simulink library "ConverterLibrary"  (R2026a)
settings: Solver=VariableStepAuto
undefined symbols (not defined in the file or in its folder): DiscIntNeverNeededParam, dspblkCoreblockFVToolHelper, gcbh, gridInverter
libraries: fl_lib x240, nesl_utility x221, ee_lib x208, slpidlib x28, eeGeneralControl x12, simulink x9, eeTransforms x4, simulink_extras x1, eePowerMeasurement x1
(part 4 of 30)

== system ConverterLibrary/Power Converter Plant/Soft-Switching Converters ==
  CLLC Converter : Subsystem  mask(CLLC Converter Plant){modelOption=Simplified, C1=6.9269e-7, C1_unit=F, Rcr1=0.001, Rcr1_unit=Ohm, C2=7.487e-7, C2_unit=F, Rcr2=0.001, Rcr2_unit=Ohm, Llk1=3.6568e-6, Llk1_unit=H, R1=0.01, R1_unit=Ohm, Llk2=3.3829e-6, Llk2_unit=H, R2=0.01, R2_unit=Ohm, Lm=5.4852e-5, Lm_unit=H, N1=30, N2=29, Co=1.0667e-3, Co_unit=F, Rco=0.02, Rco_unit=Ohm, Vco=350, Vco_unit=V, PrimaryDeviceOption=MOSFET (Ideal, Switching) with Thermal, PrimaryRon=0.001, PrimaryRon_unit=Ohm, PrimaryGoff=1e-5, PrimaryGoff_unit=1/Ohm, PrimaryVth=2.5, PrimaryVth_unit=V, PrimaryVbodydiodeOn=0.6, PrimaryVbodydiodeOn_unit=V, PrimaryRbodydiodeOn=0.001, PrimaryRbodydiodeOn_unit=Ohm, PrimaryGbodydiodeOff=1e-5, PrimaryGbodydiodeOff_unit=1/Ohm, PrimaryCparasitic=2e-10, PrimaryCparasitic_unit=F, SecondaryDeviceOption=MOSFET (Ideal, Switching) with Thermal, SecondaryRon=0.001, SecondaryRon_unit=Ohm, SecondaryGoff=1e-5, SecondaryGoff_unit=1/Ohm, SecondaryVth=2.5, SecondaryVth_unit=V, SecondaryVbodydiodeOn=0.6, SecondaryVbodydiodeOn_unit=V, SecondaryRbodydiodeOn=0.001, SecondaryRbodydiodeOn_unit=Ohm, SecondaryGbodydiodeOff=1e-5, SecondaryGbodydiodeOff_unit=1/Ohm, SecondaryCparasitic=2e-10, SecondaryCparasitic_unit=F, PrimarySimTemp=25, PrimarySimTemp_unit=degC, SecondarySimTemp=25, SecondarySimTemp_unit=degC}
      mask prompts: modelOption "Model option"; C1 "Primary resonant capacitance (C1)"; Rcr1 "Primary resonant capacitor ESR (Rcr1)"; C2 "Secondary resonant capacitance (C2)"; Rcr2 "Secondary resonant capacitor ESR (Rcr2)"; Llk1 "Primary leakage inductance (Llk1)"; R1 "Primary resistance (R1)"; Llk2 "Secondary leakage inductance (Llk2)"; R2 "Secondary resistance (R2)"; Lm "Magnetizing inductance (Lm)"; N1 "Transformer primary number of turns (N1)"; N2 "Transformer secondary number of turns (N2)"; Co "Secondary output capacitance (Co)"; Rco "Secondary output capacitance ESR (Rco)"; Vco "Initial output capacitor voltage"; PrimaryDeviceOption "Select the primary switching device"; PrimaryRon "On-state resistance"; PrimaryGoff "Off-state conductance"; PrimaryVth "Threshold voltage"; PrimaryVbodydiodeOn "Body diode forward voltage"; PrimaryRbodydiodeOn "Body diode on-resistance"; PrimaryGbodydiodeOff "Body diode off-conductance"; PrimaryCparasitic "MOSFET parasitic capacitance"; SecondaryDeviceOption "Select the secondary switching device"; SecondaryRon "On-state resistance"; SecondaryGoff "Off-state conductance"; SecondaryVth "Threshold voltage"; SecondaryVbodydiodeOn "Body diode forward voltage"; SecondaryRbodydiodeOn "Body diode on-resistance"; SecondaryGbodydiodeOff "Body diode off-conductance"; SecondaryCparasitic "MOSFET parasitic capacitance"; PrimarySimTemp "Simulation temperature"; SecondarySimTemp "Simulation temperature"
      mask help: This block models the power circuit of the CLLC resonant converter. You can choose between different semicondcutor switch model for primary and secondaryconverter. You can choose between ideal semiconductor switch, MOSFET without thermal port and tabulated MOSFET with thermal port.
      mask init:
      | %% Unit conversion: convert displayed values to base SI units
      | convMap = containers.Map( ...
      |     {'W','kW','MW','V','kV','mV','F','mF','uF','nF','pF', ...
      |      'H','mH','uH','nH','Ohm','kOhm','mOhm','S','mS','1/Ohm'}, ...
      |     {1, 1e3, 1e6, 1, 1e3, 1e-3, 1, 1e-3, 1e-6, 1e-9, 1e-12, ...
      |      1, 1e-3, 1e-6, 1e-9, 1, 1e3, 1e-3, 1, 1e-3, 1});
      | C1 = C1 * convMap(C1_unit);
      | Rcr1 = Rcr1 * convMap(Rcr1_unit);
      | C2 = C2 * convMap(C2_unit);
      | Rcr2 = Rcr2 * convMap(Rcr2_unit);
      | Llk1 = Llk1 * convMap(Llk1_unit);
      | R1 = R1 * convMap(R1_unit);
      | Llk2 = Llk2 * convMap(Llk2_unit);
      | R2 = R2 * convMap(R2_unit);
      | Lm = Lm * convMap(Lm_unit);
      | Co = Co * convMap(Co_unit);
      | Rco = Rco * convMap(Rco_unit);
      | Vco = Vco * convMap(Vco_unit);
      | PrimaryRon = PrimaryRon * convMap(PrimaryRon_unit);
      | PrimaryGoff = PrimaryGoff * convMap(PrimaryGoff_unit);
      | PrimaryVth = PrimaryVth * convMap(PrimaryVth_unit);
      | PrimaryVbodydiodeOn = PrimaryVbodydiodeOn * convMap(PrimaryVbodydiodeOn_unit);
      | PrimaryRbodydiodeOn = PrimaryRbodydiodeOn * convMap(PrimaryRbodydiodeOn_unit);
      | PrimaryGbodydiodeOff = PrimaryGbodydiodeOff * convMap(PrimaryGbodydiodeOff_unit);
      | PrimaryCparasitic = PrimaryCparasitic * convMap(PrimaryCparasitic_unit);
      | SecondaryRon = SecondaryRon * convMap(SecondaryRon_unit);
      | SecondaryGoff = SecondaryGoff * convMap(SecondaryGoff_unit);
      | SecondaryVth = SecondaryVth * convMap(SecondaryVth_unit);
      | SecondaryVbodydiodeOn = SecondaryVbodydiodeOn * convMap(SecondaryVbodydiodeOn_unit);
      | SecondaryRbodydiodeOn = SecondaryRbodydiodeOn * convMap(SecondaryRbodydiodeOn_unit);
      | SecondaryGbodydiodeOff = SecondaryGbodydiodeOff * convMap(SecondaryGbodydiodeOff_unit);
      | SecondaryCparasitic = SecondaryCparasitic * convMap(SecondaryCparasitic_unit);
      | % Simulation temperature (primary bridge, thermal MOSFETs)
      | % Temperature is an OFFSET unit (K = degC + 273.15), so it cannot use the
      | % multiplicative convMap above; convert it explicitly. PrimarySimTemp_K is read directly
      | % by each primary thermal MOSFET junction-temperature initial target and by every
      | % Temperature Source in the primary bridge.
      | if strcmp(PrimarySimTemp_unit, 'degC')
      |     PrimarySimTemp_K = PrimarySimTemp + 273.15;
      | elseif strcmp(PrimarySimTemp_unit, 'K')
      |     PrimarySimTemp_K = PrimarySimTemp;
      | else
      |     error('CLLC Converter Power Circuit: unrecognized simulation-temperature unit "%s" (expected degC or K).', PrimarySimTemp_unit);
      | end
      | % Simulation temperature (secondary bridge, thermal MOSFETs)
      | % Temperature is an OFFSET unit (K = degC + 273.15), so it cannot use the
      | % multiplicative convMap above; convert it explicitly. SecondarySimTemp_K is read directly
      | % by each secondary thermal MOSFET junction-temperature initial target and by every
      | % Temperature Source in the secondary bridge.
      | if strcmp(SecondarySimTemp_unit, 'degC')
      |     SecondarySimTemp_K = SecondarySimTemp + 273.15;
      | elseif strcmp(SecondarySimTemp_unit, 'K')
      |     SecondarySimTemp_K = SecondarySimTemp;
      | else
      |     error('CLLC Converter Power Circuit: unrecognized simulation-temperature unit "%s" (expected degC or K).', SecondarySimTemp_unit);
      | end
      settings: CopyFcn="set_param(gcbh,\"LinkStatus\",\"none\");"  PortSchema="{\"entries\":[{\"content\":{\"sides\":[{\"content\":{\"connectorIds\":[\"LConn1\",\"LConn2\"]},\"type\":\"ConnectorPlacement.EquallySpacedRectSide\",\"uuid\":\"0e984043-8111-4613-9feb-f4d4d19f792a\"},{\"content\":{\"connectorIds\":[\"RConn1\",\"RConn2\"],\"side\":\"RIGHT\"},\"type\":\"ConnectorPlacement.EquallySpacedRectSide\",\"uuid\":\"aee9207a-aaf7-4114-a348-153041cb19a5\"},{\"content\":{\"connectorIds\":[\"In1\",\"Out1\",\"In2\"],\"side\":\"TOP\"},\"type\":\"ConnectorPlacement.EquallySpacedRectSide\",\"uuid\":\"cf17a722-cb18-4642-bf19-4f4ee8ce3a25\"}]},\"type\":\"ConnectorPlacement.EquallySpacedConnector\",\"uuid\":\"0a50e5d5-a4bf-4817-9816-42fb9bad860d\"}],\"packageUris\":[\"http://schema.mathworks.com/mf0/Connector/R2020b\"],\"version\":\"1.0\"}"
      mask Help: web('CLLCPowerCircuit.html')
      mask TypeOptions modelOption: Simplified | Detailed
      mask Callback modelOption: selectCLLCConverterModelOption(gcb);
      mask TypeOptions C1_unit: F | mF | uF | nF | pF
      mask TypeOptions Rcr1_unit: Ohm | kOhm | mOhm
      mask TypeOptions C2_unit: F | mF | uF | nF | pF
      mask TypeOptions Rcr2_unit: Ohm | kOhm | mOhm
      mask TypeOptions Llk1_unit: H | mH | uH | nH
      mask TypeOptions R1_unit: Ohm | kOhm | mOhm
      mask TypeOptions Llk2_unit: H | mH | uH | nH
      mask TypeOptions R2_unit: Ohm | kOhm | mOhm
      mask TypeOptions Lm_unit: H | mH | uH | nH
      mask TypeOptions Co_unit: F | mF | uF | nF | pF
      mask TypeOptions Rco_unit: Ohm | kOhm | mOhm
      mask TypeOptions Vco_unit: V | kV | mV
      mask TypeOptions PrimaryDeviceOption: Ideal Switch | MOSFET (Ideal, Switching) with Thermal
      mask Callback PrimaryDeviceOption: selectCLLCPrimaryMOSFET(gcb);
      mask TypeOptions PrimaryRon_unit: Ohm | kOhm | mOhm
      mask TypeOptions PrimaryGoff_unit: 1/Ohm | S | mS
      mask TypeOptions PrimaryVth_unit: V | kV | mV
      mask TypeOptions PrimaryVbodydiodeOn_unit: V | mV
      mask TypeOptions PrimaryRbodydiodeOn_unit: Ohm | kOhm | mOhm
      mask TypeOptions PrimaryGbodydiodeOff_unit: 1/Ohm | S | mS
      mask TypeOptions PrimaryCparasitic_unit: F | mF | uF | nF | pF
      mask TypeOptions SecondaryDeviceOption: Ideal Switch | MOSFET (Ideal, Switching) with Thermal
      mask Callback SecondaryDeviceOption: selectCLLCSecondaryMOSFET(gcb);
      mask TypeOptions SecondaryRon_unit: Ohm | kOhm | mOhm
      mask TypeOptions SecondaryGoff_unit: 1/Ohm | S | mS
      mask TypeOptions SecondaryVth_unit: V | kV | mV
      mask TypeOptions SecondaryVbodydiodeOn_unit: V | mV
      mask TypeOptions SecondaryRbodydiodeOn_unit: Ohm | kOhm | mOhm
      mask TypeOptions SecondaryGbodydiodeOff_unit: 1/Ohm | S | mS
      mask TypeOptions SecondaryCparasitic_unit: F | mF | uF | nF | pF
      mask TypeOptions PrimarySimTemp_unit: degC | K
      mask TypeOptions SecondarySimTemp_unit: degC | K
      mask DialogControl ParameterGroupVar Prompt: CLLC Resonant Converter Plant
      mask DialogControl CLLCTank Prompt: CLLC converter parameters
      mask DialogControl TransformerParameters Prompt: Transformer
      mask DialogControl PrimarySwitch Prompt: Primary semiconductor switch
      mask DialogControl PrimaryOpenMOSFETMask Prompt: Open the MOSFET block mask
      mask DialogControl PrimaryOpenMOSFETMask Callback: openCLLCDeviceMask(gcb, 'primaryThermalMOSFET');
      mask DialogControl PrimaryApplyMOSFETParam Prompt: Apply parameters to all primary MOSFET blocks
      mask DialogControl PrimaryApplyMOSFETParam Callback: applyCLLCDeviceParameters(gcb, 'primaryThermalMOSFET');
      mask DialogControl SecondarySwitch Prompt: Secondary semiconductor switch
      mask DialogControl SecondaryOpenMOSFETMask Prompt: Open the MOSFET block mask
      mask DialogControl SecondaryOpenMOSFETMask Callback: openCLLCDeviceMask(gcb, 'secondaryThermalMOSFET');
      mask DialogControl SecondaryApplyMOSFETParam Prompt: Apply parameters to all secondary MOSFET blocks
      mask DialogControl SecondaryApplyMOSFETParam Callback: applyCLLCDeviceParameters(gcb, 'secondaryThermalMOSFET');
      mask DialogControl ExportPanel Prompt: Export to Unmasked Subsystem
      mask DialogControl ExportInfo Prompt: To customize the converter, export it as an unmasked subsystem with the active variant flattened - a standalone, fully-editable circuit plus a parameter file. Requires the "Variant Manager for Simulink" add-on.
      mask DialogControl exportToModel Prompt: Export
      mask DialogControl exportToModel Callback: exportConverterModelFromMask(gcb);
      mask Display: image('CLLCConverterIcon.svg');
  DAB Converter : Subsystem  mask(Dual Active Bridge DC-DC Converter){modelOption=Detailed, ratedPower=10000, ratedPower_unit=W, Vin=750, Vin_unit=V, Vout=525, Vout_unit=V, Fsw=100000, Fsw_unit=Hz, turnsRatio=1.4286, Co=2.963e-5, Co_unit=F, Rco=1, Rco_unit=mOhm, seriesInductorOption=Use transformer leakage inductance, Lr=0, Lr_unit=H, RLr=0.01, RLr_unit=Ohm, Lm=1.4062e-3, Lm_unit=H, Llk1=3.913e-5, Llk1_unit=H, RLlk1=0.01, RLlk1_unit=Ohm, Llk2=4.7935e-6, Llk2_unit=H, RLlk2=0.01, RLlk2_unit=Ohm, Vco=525, Vco_unit=V, switchDeviceOptionPri=MOSFET (Ideal, Switching) with Thermal, RdsOnPri=0.005, RdsOnPri_unit=Ohm, GdsOffPri=1e-5, GdsOffPri_unit=1/Ohm, VthPri=3, VthPri_unit=V, CossPri=2e-10, CossPri_unit=F, simTempPri=25, simTempPri_unit=degC, VfPri=0.005, VfPri_unit=V, RdPri=1, RdPri_unit=mOhm, GdPri=1e-5, GdPri_unit=1/Ohm, switchDeviceOptionSec=MOSFET (Ideal, Switching) with Thermal, RdsOnSec=0.005, RdsOnSec_unit=Ohm, GdsOffSec=1e-5, GdsOffSec_unit=1/Ohm, VthSec=3, VthSec_unit=V, CossSec=2e-10, CossSec_unit=F, simTempSec=25, simTempSec_unit=degC, VfSec=0.005, VfSec_unit=V, RdSec=1, RdSec_unit=mOhm, GdSec=1e-5, GdSec_unit=1/Ohm}
      mask prompts: modelOption "Model option"; ratedPower "Rated power"; Vin "Nominal input voltage"; Vout "Nominal output voltage"; Fsw "Switching frequency"; turnsRatio "Transformer turns ratio (Np/Ns)"; Co "Secondary output capacitance"; Rco "Secondary output capacitance ESR"; seriesInductorOption "Series inductance"; Lr "Series inductance (Lr)"; RLr "Series inductance resistance"; Lm "Magnetizing inductance (Lm)"; Llk1 "Primary leakage inductance (Llk1)"; RLlk1 "Primary winding resistance"; Llk2 "Secondary leakage inductance (Llk2)"; RLlk2 "Secondary winding resistance"; Vco "Initial output capacitor voltage"; switchDeviceOptionPri "Switch device"; RdsOnPri "On-state resistance (RdsOn)"; GdsOffPri "Off-state conductance (GdsOff)"; VthPri "Threshold voltage"; CossPri "Output capacitance (Coss)"; simTempPri "Simulation temperature"; VfPri "Diode forward voltage (Vf)"; RdPri "Diode on resistance (Rd)"; GdPri "Diode off conductance (Gd)"; switchDeviceOptionSec "Switch device"; RdsOnSec "On-state resistance (RdsOn)"; GdsOffSec "Off-state conductance (GdsOff)"; VthSec "Threshold voltage"; CossSec "Output capacitance (Coss)"; simTempSec "Simulation temperature"; VfSec "Diode forward voltage (Vf)"; RdSec "Diode on resistance (Rd)"; GdSec "Diode off conductance (Gd)"
      mask help: Dual Active Bridge (DAB) DC-DC Converter with variant options for HDL and Simulation models.
      mask init:
      | %% Unit conversion: convert displayed values to base SI units
      | convMap = containers.Map( ...
      |     {'W','kW','MW','V','kV','mV','F','mF','uF','nF','pF', ...
      |      'H','mH','uH','nH','Ohm','kOhm','mOhm','S','mS','1/Ohm', ...
      |      'Hz','kHz','MHz'}, ...
      |     {1, 1e3, 1e6, 1, 1e3, 1e-3, 1, 1e-3, 1e-6, 1e-9, 1e-12, ...
      |      1, 1e-3, 1e-6, 1e-9, 1, 1e3, 1e-3, 1, 1e-3, 1, ...
      |      1, 1e3, 1e6});
      | 
      | ratedPower_SI = ratedPower * convMap(ratedPower_unit);
      | Vin_SI = Vin * convMap(Vin_unit);
      | Vout_SI = Vout * convMap(Vout_unit);
      | Fsw_SI = Fsw * convMap(Fsw_unit);
      | Llk1_SI = Llk1 * convMap(Llk1_unit);
      | RLlk1_SI = RLlk1 * convMap(RLlk1_unit);
      | Llk2_SI = Llk2 * convMap(Llk2_unit);
      | RLlk2_SI = RLlk2 * convMap(RLlk2_unit);
      | Lr_SI = Lr * convMap(Lr_unit);
      | RLr_SI = RLr * convMap(RLr_unit);
      | % When the model compiles, the transformer leakages must be positive, and so must Lr when the
      | % external inductor is used. A dialog change is not checked, so Lr can be entered after the option.
      | if any(strcmp(get_param(bdroot(gcb), 'SimulationStatus'), {'updating', 'initializing'}))
      |     if ~(isfinite(Llk1_SI) && Llk1_SI > 0 && isfinite(Llk2_SI) && Llk2_SI > 0)
      |         error('The transformer leakage inductances must be positive. Primary: %g H, secondary: %g H.', Llk1_SI, Llk2_SI);
      |     end
      |     if strcmp(get_param(gcb, 'seriesInductorOption'), 'Use external inductance') && ~(isfinite(Lr_SI) && Lr_SI > 0)
      |         error('The external series inductance must be positive when it is used. Lr: %g H.', Lr_SI);
      |     end
      | end
      | Lm_SI = Lm * convMap(Lm_unit);
      | Co_SI = Co * convMap(Co_unit);
      | Rco_SI = Rco * convMap(Rco_unit);
      | Vco_SI = Vco * convMap(Vco_unit);
      | 
      | %% Primary switch params
      | RdsOnPri_SI = RdsOnPri * convMap(RdsOnPri_unit);
      | GdsOffPri_SI = GdsOffPri * convMap(GdsOffPri_unit);
      | VthPri_SI = VthPri * convMap(VthPri_unit);
      | CossPri_SI = CossPri * convMap(CossPri_unit);
      | 
      | %% Secondary switch params
      | RdsOnSec_SI = RdsOnSec * convMap(RdsOnSec_unit);
      | GdsOffSec_SI = GdsOffSec * convMap(GdsOffSec_unit);
      | VthSec_SI = VthSec * convMap(VthSec_unit);
      | CossSec_SI = CossSec * convMap(CossSec_unit);
      | 
      | %% Primary switch protection-diode params
      | VfPri_SI = VfPri * convMap(VfPri_unit);
      | RdPri_SI = RdPri * convMap(RdPri_unit);
      | GdPri_SI = GdPri * convMap(GdPri_unit);
      | 
      | %% Secondary switch protection-diode params
      | VfSec_SI = VfSec * convMap(VfSec_unit);
      | RdSec_SI = RdSec * convMap(RdSec_unit);
      | GdSec_SI = GdSec * convMap(GdSec_unit);
      | 
      | 
      | %% Simulation temperature (thermal MOSFET)
      | % Temperature is an OFFSET unit (K = degC + 273.15), so it cannot use the
      | % multiplicative convMap; convert it explicitly. These Kelvin variables are
      | % read directly by each thermal MOSFET device junction-temperature target and
      | % by each bridge Temperature Source.
      | if strcmp(simTempPri_unit, 'degC')
      |     simTempPri_K = simTempPri + 273.15;
      | else
      |     simTempPri_K = simTempPri;
      | end
      | if strcmp(simTempSec_unit, 'degC')
      |     simTempSec_K = simTempSec + 273.15;
      | else
      |     simTempSec_K = simTempSec;
      | end
      | 
      | %% Apply variant selection
      | selectDABConverterModelOption(gcb);
      settings: CopyFcn="set_param(gcbh,\"LinkStatus\",\"none\");"  PortSchema="{\"entries\":[{\"content\":{\"sides\":[{\"content\":{\"connectorIds\":[\"LConn1\",\"LConn2\"]},\"type\":\"ConnectorPlacement.EquallySpacedRectSide\",\"uuid\":\"5eb81d01-b33d-480d-b92b-9ee197a9667d\"},{\"content\":{\"connectorIds\":[\"RConn1\",\"RConn2\"],\"side\":\"RIGHT\"},\"type\":\"ConnectorPlacement.EquallySpacedRectSide\",\"uuid\":\"a719554b-e33a-474b-8c80-408706add5ae\"},{\"content\":{\"connectorIds\":[\"In1\",\"Out1\",\"In2\"],\"side\":\"TOP\"},\"type\":\"ConnectorPlacement.EquallySpacedRectSide\",\"uuid\":\"aea510b9-aefe-49d3-b91f-0f6ebd0a6b41\"}]},\"type\":\"ConnectorPlacement.EquallySpacedConnector\",\"uuid\":\"00bcdd44-1110-449b-876a-23d9733cbf45\"}],\"packageUris\":[\"http://schema.mathworks.com/mf0/Connector/R2020b\"],\"version\":\"1.0\"}"
      mask Help: web('DABConverter.html')
      mask TypeOptions modelOption: Simplified | Detailed
      mask Callback modelOption: selectDABConverterModelOption(gcb);
      mask TypeOptions ratedPower_unit: W | kW | MW
      mask TypeOptions Vin_unit: mV | V | kV
      mask TypeOptions Vout_unit: mV | V | kV
      mask TypeOptions Fsw_unit: Hz | kHz | MHz
      mask TypeOptions Co_unit: F | mF | uF | nF | pF
      mask TypeOptions Rco_unit: mOhm | Ohm | kOhm
      mask TypeOptions seriesInductorOption: Use external inductance | Use transformer leakage inductance
      mask Callback seriesInductorOption: selectDABSeriesInductor(gcb);
      mask TypeOptions Lr_unit: H | mH | uH | nH
      mask TypeOptions RLr_unit: mOhm | Ohm | kOhm
      mask TypeOptions Lm_unit: H | mH | uH | nH
      mask TypeOptions Llk1_unit: H | mH | uH | nH
      mask TypeOptions RLlk1_unit: mOhm | Ohm | kOhm
      mask TypeOptions Llk2_unit: H | mH | uH | nH
      mask TypeOptions RLlk2_unit: mOhm | Ohm | kOhm
      mask TypeOptions Vco_unit: V | kV | mV
      mask TypeOptions switchDeviceOptionPri: Ideal Switch | MOSFET (Ideal, Switching) with Thermal
      mask Callback switchDeviceOptionPri: selectDABConverterSwitchDevice(gcb)
      mask TypeOptions RdsOnPri_unit: mOhm | Ohm | kOhm
      mask TypeOptions GdsOffPri_unit: S | mS | 1/Ohm
      mask TypeOptions VthPri_unit: mV | V | kV
      mask TypeOptions CossPri_unit: F | mF | uF | nF | pF
      mask TypeOptions simTempPri_unit: degC | K
      mask TypeOptions VfPri_unit: mV | V | kV
      mask TypeOptions RdPri_unit: mOhm | Ohm | kOhm
      mask TypeOptions GdPri_unit: S | mS | 1/Ohm
      mask TypeOptions switchDeviceOptionSec: Ideal Switch | MOSFET (Ideal, Switching) with Thermal
      mask Callback switchDeviceOptionSec: selectDABConverterSwitchDevice(gcb)
      mask TypeOptions RdsOnSec_unit: mOhm | Ohm | kOhm
      mask TypeOptions GdsOffSec_unit: S | mS | 1/Ohm
      mask TypeOptions VthSec_unit: mV | V | kV
      mask TypeOptions CossSec_unit: F | mF | uF | nF | pF
      mask TypeOptions simTempSec_unit: degC | K
      mask TypeOptions VfSec_unit: mV | V | kV
      mask TypeOptions RdSec_unit: mOhm | Ohm | kOhm
      mask TypeOptions GdSec_unit: S | mS | 1/Ohm
      mask DialogControl DABConverterParameters Prompt: DAB Converter Parameters
      mask DialogControl TransformerParameters Prompt: Transformer
      mask DialogControl PrimarySwitch Prompt: Primary Switch
      mask DialogControl openMOSFETPriMask Prompt: Open MOSFET block mask
      mask DialogControl openMOSFETPriMask Callback: open_system([gcb '/DABConverterVariant/DetailedModel/PrimaryBridge/SwitchingMOSFETwithThermal/MOSFETPriA1'], 'mask')
      mask DialogControl applyMOSFETPriParam Prompt: Apply parameters to all primary MOSFET blocks
      mask DialogControl applyMOSFETPriParam Callback: applyDABConverterMOSFETParameters(gcb, 'primary')
      mask DialogControl SecondarySwitch Prompt: Secondary Switch
      mask DialogControl openMOSFETSecMask Prompt: Open MOSFET block mask
      mask DialogControl openMOSFETSecMask Callback: open_system([gcb '/DABConverterVariant/DetailedModel/SecondaryBridge/SwitchingMOSFETwithThermal/MOSFETSecA1'], 'mask')
      mask DialogControl applyMOSFETSecParam Prompt: Apply parameters to all secondary MOSFET blocks
      mask DialogControl applyMOSFETSecParam Callback: applyDABConverterMOSFETParameters(gcb, 'secondary')
      mask DialogControl ExportPanel Prompt: Export to Unmasked Subsystem
      mask DialogControl ExportInfo Prompt: To customize the converter, export it as an unmasked subsystem with the active variant flattened - a standalone, fully-editable circuit plus a parameter file. Requires the "Variant Manager for Simulink" add-on.
      mask DialogControl exportToModel Prompt: Export
      mask DialogControl exportToModel Callback: exportConverterModelFromMask(gcb);
      mask Display: image('DABConverterIcon.svg');
  LLC Converter : Subsystem  mask(LLC Converter Plant){llcConverterModel=Detailed Full-Bridge, ratedPower=10e3, ratedPower_unit=W, VIn=380, VIn_unit=V, Cr=3.3703e-7, Cr_unit=F, seriesInductorOption=Use transformer leakage inductance, Lr=30, Lr_unit=uH, RLr=1, RLr_unit=mOhm, Llk1=7.14e-6, Llk1_unit=H, R1=0.01, R1_unit=Ohm, Llk2=4.0645e-7, Llk2_unit=H, R2=0.01, R2_unit=Ohm, Lm=9.7705e-5, Lm_unit=H, n=9.6154e-1, Cf=7.1111e-4, Cf_unit=F, Esr=0.02, Esr_unit=Ohm, Vco=350, Vco_unit=V, primaryDeviceOption=Ideal Semiconductor Switch, RdsOn=0.001, RdsOn_unit=Ohm, GdsOff=1e-5, GdsOff_unit=1/Ohm, Vth=2.5, Vth_unit=V, VfBody=0.6, VfBody_unit=V, RdBody=0.001, RdBody_unit=Ohm, GdBody=1e-5, GdBody_unit=1/Ohm, Cdsparasitic=2e-10, Cdsparasitic_unit=F, simTempPri=25, simTempPri_unit=degC, rectifierOption=Full Bridge, secondaryDeviceOption=Ideal Diode, VfSec=0.6, VfSec_unit=V, RdSec=0.001, RdSec_unit=Ohm, GdSec=1e-5, GdSec_unit=1/Ohm, simTempSec=25, simTempSec_unit=degC}
      mask prompts: llcConverterModel "LLC Converter model"; ratedPower "Rated power (P)"; VIn "Nominal input voltage (Vdc)"; Cr "Resonant capacitance (Cr)"; seriesInductorOption "Series resonant inductance"; Lr "Series resonant inductance (Lr)"; RLr "Series inductance resistance"; Llk1 "Primary leakage inductance (Lr)"; R1 "Primary resistance (R1)"; Llk2 "Secondary leakage inductance (Llk2)"; R2 "Secondary resistance (R2)"; Lm "Magnetizing inductance (Lm)"; n "Transformer turns ratio (n)"; Cf "Output filter capacitance (Co)"; Esr "Output filter capacitor ESR (Rco)"; Vco "Initial output capacitor voltage"; primaryDeviceOption "Select the primary switching device"; RdsOn "On-state resistance"; GdsOff "Off-state conductance"; Vth "Threshold voltage"; VfBody "Body diode forward voltage"; RdBody "Body diode on-resistance"; GdBody "Body diode off-conductance"; Cdsparasitic "MOSFET parasitic capacitance"; simTempPri "Simulation temperature"; rectifierOption "Select the rectifier topology"; secondaryDeviceOption "Select the secondary diode"; VfSec "Forward voltage"; RdSec "On resistance"; GdSec "Off conductance"; simTempSec "Simulation temperature"
      mask help: This block models the power circuit of the LLC resonant converter. You can choose between different switch and diode models. For the primary semiconductor switch, you can choose between ideal semiconductor switch, MOSFET without thermal port and tabulated MOSFET with thermal port. For the secondary, you can choose between ideal and tabulated diode.
      mask init:
      | %% Unit conversion: convert displayed values to base SI units
      | convMap = containers.Map( ...
      |     {'W','kW','MW','V','kV','mV','F','mF','uF','nF','pF', ...
      |      'H','mH','uH','nH','Ohm','kOhm','mOhm','S','mS','1/Ohm'}, ...
      |     {1, 1e3, 1e6, 1, 1e3, 1e-3, 1, 1e-3, 1e-6, 1e-9, 1e-12, ...
      |      1, 1e-3, 1e-6, 1e-9, 1, 1e3, 1e-3, 1, 1e-3, 1});
      | ratedPower = ratedPower * convMap(ratedPower_unit);
      | VIn = VIn * convMap(VIn_unit);
      | Cr = Cr * convMap(Cr_unit);
      | Lr_SI = Lr * convMap(Lr_unit);
      | RLr_SI = RLr * convMap(RLr_unit);
      | Llk1 = Llk1 * convMap(Llk1_unit);
      | R1 = R1 * convMap(R1_unit);
      | Llk2 = Llk2 * convMap(Llk2_unit);
      | R2 = R2 * convMap(R2_unit);
      | Lm = Lm * convMap(Lm_unit);
      | Cf = Cf * convMap(Cf_unit);
      | Esr = Esr * convMap(Esr_unit);
      | Vco_SI = Vco * convMap(Vco_unit);
      | RdsOn = RdsOn * convMap(RdsOn_unit);
      | GdsOff = GdsOff * convMap(GdsOff_unit);
      | Vth = Vth * convMap(Vth_unit);
      | VfBody = VfBody * convMap(VfBody_unit);
      | RdBody = RdBody * convMap(RdBody_unit);
      | GdBody = GdBody * convMap(GdBody_unit);
      | Cdsparasitic = Cdsparasitic * convMap(Cdsparasitic_unit);
      | VfSec = VfSec * convMap(VfSec_unit);
      | RdSec = RdSec * convMap(RdSec_unit);
      | GdSec = GdSec * convMap(GdSec_unit);
      | %% Transformer turns ratio and leakage inductances
      | % A centre-tap rectifier halves the ratio and doubles the secondary leakage of the
      | % centre-tapped transformer. With an external series inductor the leakages are a small
      | % share of it, referred to each winding, so they are never zero.
      | leakageShareOfExternalInductor = 1e-3;
      | primaryLeakage = Llk1;
      | secondaryLeakage = Llk2;
      | % Read by name: seriesInductorOption is an evaluated popup, so its workspace value is an index
      | if strcmp(get_param(gcb, 'seriesInductorOption'), 'Use external inductance') && startsWith(get_param(gcb, 'llcConverterModel'), 'Detailed')
      |     primaryLeakage = leakageShareOfExternalInductor*Lr_SI;
      |     secondaryLeakage = leakageShareOfExternalInductor*Lr_SI/n^2;
      | end
      | if ~(isfinite(primaryLeakage) && primaryLeakage > 0 && isfinite(secondaryLeakage) && secondaryLeakage > 0)
      |     error('The transformer leakage inductances must be positive. Primary: %g H, secondary: %g H.', ...
      |         primaryLeakage, secondaryLeakage);
      | end
      | if strcmp(rectifierOption, 'Centre-Tap')
      |     xfmrTurnsRatio = n/2;
      |     xfmrSecondaryLeakage = 2*secondaryLeakage;
      | else
      |     xfmrTurnsRatio = n;
      |     xfmrSecondaryLeakage = secondaryLeakage;
      | end
      | xfmrPrimaryLeakage = primaryLeakage;
      | %% Simulation temperature (loss-only, thermal MOSFET device)
      | % Temperature is an OFFSET unit (K = degC + 273.15), so it cannot use the
      | % multiplicative convMap above; convert it explicitly. simTempPri_K is read
      | % directly by each thermal MOSFET's junction-temperature initial target and by
      | % each Temperature Source in the primary bridge.
      | if strcmp(simTempPri_unit, 'degC')
      |     simTempPri_K = simTempPri + 273.15;
      | elseif strcmp(simTempPri_unit, 'K')
      |     simTempPri_K = simTempPri;
      | else
      |     error('LLC Converter Power Circuit: unrecognized simulation-temperature unit "%s" (expected degC or K).', simTempPri_unit);
      | end
      | %% Simulation temperature (secondary rectifier, tabulated diode)
      | % Same offset-unit conversion as the primary above (K = degC + 273.15), which is why
      | % neither can use the multiplicative convMap. simTempSec_K is read by every tabulated
      | % rectifier diode's device simulation temperature. That is the only temperature input
      | % those blocks have: in this configuration the diode has two electrical ports and no
      | % thermal port, so a junction-temperature target on it would be inert.
      | if strcmp(simTempSec_unit, 'degC')
      |     simTempSec_K = simTempSec + 273.15;
      | elseif strcmp(simTempSec_unit, 'K')
      |     simTempSec_K = simTempSec;
      | else
      |     error('LLC Converter Power Circuit: unrecognized simulation-temperature unit "%s" (expected degC or K).', simTempSec_unit);
      | end
      | %% Select model variant and visibility
      | selectLLCPlantModel(gcb);
      | %% Block icon
      | % The icon is drawn by the mask Display code, which resolves its four artwork files
      | % (FullBridgeLLCCentreTapRectifier.svg and siblings) by name from the MATLAB path.
      | % They live in Components/ConverterPlants/CombinedLLCConverterPlant/icons, which
      | % the project puts on the path. An earlier design kept the SVG source in
      | % model-workspace variables and unpacked it to tempdir here; those variables no longer
      | % exist, so that code only stranded a file handle on a zero-byte temp file every run.
      settings: CopyFcn="set_param(gcbh,\"LinkStatus\",\"none\");"  PortSchema="{\"entries\":[{\"content\":{\"sides\":[{\"content\":{\"connectorIds\":[\"LConn1\",\"LConn2\"]},\"type\":\"ConnectorPlacement.EquallySpacedRectSide\",\"uuid\":\"7d0af355-cbc1-43de-86a8-478c0417a0e6\"},{\"content\":{\"connectorIds\":[\"RConn1\",\"RConn2\"],\"side\":\"RIGHT\"},\"type\":\"ConnectorPlacement.EquallySpacedRectSide\",\"uuid\":\"e5e2e9fd-b3a0-4f29-84de-d1d266c8101b\"},{\"content\":{\"connectorIds\":[\"In1\",\"Out1\"],\"side\":\"TOP\"},\"type\":\"ConnectorPlacement.EquallySpacedRectSide\",\"uuid\":\"2a0404a0-819d-4dd0-9f33-52ca4a6707b9\"}]},\"type\":\"ConnectorPlacement.EquallySpacedConnector\",\"uuid\":\"862cc0c4-78b7-4235-be37-b455f1ccafcc\"}],\"packageUris\":[\"http://schema.mathworks.com/mf0/Connector/R2020b\"],\"version\":\"1.0\"}"
      mask Help: web('LLCConverterPlant.html')
      mask TypeOptions llcConverterModel: Simplified Half-Bridge | Detailed Half-Bridge | Detailed Full-Bridge
      mask Callback llcConverterModel: selectLLCPlantModel(gcb);
      mask TypeOptions ratedPower_unit: W | kW | MW
      mask TypeOptions VIn_unit: V | kV | mV
      mask TypeOptions Cr_unit: F | mF | uF | nF | pF
      mask TypeOptions seriesInductorOption: Use external inductance | Use transformer leakage inductance
      mask Callback seriesInductorOption: selectLLCSeriesInductor(gcb);
      mask TypeOptions Lr_unit: H | mH | uH | nH
      mask TypeOptions RLr_unit: Ohm | mOhm | kOhm
      mask TypeOptions Llk1_unit: H | mH | uH | nH
      mask TypeOptions R1_unit: Ohm | kOhm | mOhm
      mask TypeOptions Llk2_unit: H | mH | uH | nH
      mask TypeOptions R2_unit: Ohm | kOhm | mOhm
      mask TypeOptions Lm_unit: H | mH | uH | nH
      mask TypeOptions Cf_unit: F | mF | uF | nF | pF
      mask TypeOptions Esr_unit: Ohm | kOhm | mOhm
      mask TypeOptions Vco_unit: V | kV | mV
      mask TypeOptions primaryDeviceOption: Ideal Semiconductor Switch | MOSFET (Ideal, Switching) with Thermal
      mask Callback primaryDeviceOption: selectLLCPlantPrimaryMOSFET(gcb);
      mask TypeOptions RdsOn_unit: Ohm | kOhm | mOhm
      mask TypeOptions GdsOff_unit: 1/Ohm | S | mS
      mask TypeOptions Vth_unit: V | kV | mV
      mask TypeOptions VfBody_unit: V | mV
      mask TypeOptions RdBody_unit: Ohm | kOhm | mOhm
      mask TypeOptions GdBody_unit: 1/Ohm | S | mS
      mask TypeOptions Cdsparasitic_unit: F | mF | uF | nF | pF
      mask TypeOptions simTempPri_unit: degC | K
      mask TypeOptions rectifierOption: Centre-Tap | Full Bridge
      mask Callback rectifierOption: selectLLCPlantSecondaryDiode(gcb);
      mask TypeOptions secondaryDeviceOption: Ideal Diode | Tabulated Diode
      mask Callback secondaryDeviceOption: selectLLCPlantSecondaryDiode(gcb);
      mask TypeOptions VfSec_unit: V | mV
      mask TypeOptions RdSec_unit: Ohm | kOhm | mOhm
      mask TypeOptions GdSec_unit: 1/Ohm | S | mS
      mask TypeOptions simTempSec_unit: degC | K
      mask DialogControl LLCTank Prompt: Resonant tank parameters
      mask DialogControl Switch Prompt: Primary Inverter
      mask DialogControl openMOSFETMask Prompt: Open the MOSFET block mask
      mask DialogControl openMOSFETMask Callback:
      | blockPath = [gcb, '/LLC Primary Inverter and Resonant Tank/LLC Detailed Model/Inverter/Primary Inverter'];
      | llcConverterChoice = get_param(gcb,'llcConverterModel');
      | switch llcConverterChoice
      |     case 'Detailed Half-Bridge'
      |         open_system([blockPath, '/Half Bridge with Thermal/MOSFETA1'], 'mask');
      |     case 'Detailed Full-Bridge'
      |         open_system([blockPath, '/Full Bridge with Thermal/MOSFETA1'], 'mask');
      |     otherwise
      |         error('Open the MOSFET mask only in a Detailed model with the thermal MOSFET device selected.');
      | end
      mask DialogControl applyMOSFETParam Prompt: Apply parameters to all primary MOSFET blocks
      mask DialogControl applyMOSFETParam Callback:
      | llcConverterChoice = get_param(gcb, 'llcConverterModel');
      | primaryInvBase = [gcb, '/LLC Primary Inverter and Resonant Tank/LLC Detailed Model/Inverter/Primary Inverter'];
      | switch llcConverterChoice
      |     case 'Detailed Half-Bridge'
      |         srcBlock = [primaryInvBase, '/Half Bridge with Thermal/MOSFETA1'];
      |         dstBlocks = {[primaryInvBase, '/Half Bridge with Thermal/MOSFETA2']};
      |     case 'Detailed Full-Bridge'
      |         srcBlock = [primaryInvBase, '/Full Bridge with Thermal/MOSFETA1'];
      |         dstBlocks = {[primaryInvBase, '/Full Bridge with Thermal/MOSFETA2'], [primaryInvBase, '/Full Bridge with Thermal/MOSFETB1'], [primaryInvBase, '/Full Bridge with Thermal/MOSFETB2']};
      |     otherwise
      |         return;
      | end
      | paramNames = fieldnames(get_param(srcBlock, 'DialogParameters'));
      | paramValues = cellfun(@(x) get_param(srcBlock, x), paramNames, 'UniformOutput', false);
      | for k = 1:numel(dstBlocks)
      |     cellfun(@(x, y) set_param(dstBlocks{k}, x, y), paramNames, paramValues, 'UniformOutput', false);
      | end
      | fprintf('Applied MOSFET parameters to %d blocks.\n', numel(dstBlocks));
      mask DialogControl Diode Prompt: Secondary Rectifier
      mask DialogControl openDiodeMask Prompt: Open the Diode block mask
      mask DialogControl openDiodeMask Callback:
      | rectBridge = [gcb, '/Rectifier/Rectifier Bridge'];
      | if strcmp(get_param(gcb, 'rectifierOption'), 'Centre-Tap')
      |     diodeBlk = [rectBridge, '/Centre-Tap Tabulated Diode/Diode1'];
      | else
      |     diodeBlk = [rectBridge, '/Full Bridge Tabulated Diode/Diode1'];
      | end
      | open_system(diodeBlk, 'mask');
      mask DialogControl applyDiodeParam Prompt: Apply parameters to all secondary Diode blocks
      mask DialogControl applyDiodeParam Callback:
      | rectBridge = [gcb, '/Rectifier/Rectifier Bridge'];
      | if strcmp(get_param(gcb, 'rectifierOption'), 'Centre-Tap')
      |     subsys = [rectBridge, '/Centre-Tap Tabulated Diode'];
      | else
      |     subsys = [rectBridge, '/Full Bridge Tabulated Diode'];
      | end
      | srcBlock = [subsys, '/Diode1'];
      | dstBlocks = find_system(subsys, 'SearchDepth', 1, 'LookUnderMasks', 'all', 'BlockType', 'SimscapeBlock');
      | dstBlocks(strcmp(dstBlocks, srcBlock)) = [];
      | dstBlocks(contains(dstBlocks, 'Open Circuit')) = [];
      | paramNames = fieldnames(get_param(srcBlock, 'DialogParameters'));
      | paramValues = cellfun(@(x) get_param(srcBlock, x), paramNames, 'UniformOutput', false);
      | for k = 1:numel(dstBlocks)
      |     cellfun(@(x, y) set_param(dstBlocks{k}, x, y), paramNames, paramValues, 'UniformOutput', false);
      | end
      | fprintf('Applied Diode1 parameters to %d other diode blocks.\\n', numel(dstBlocks));
      mask DialogControl ExportPanel Prompt: Export to Unmasked Subsystem
      mask DialogControl ExportInfo Prompt: To customize the converter, export it as an unmasked subsystem with the active variant flattened - a standalone, fully-editable circuit plus a parameter file. Requires the "Variant Manager for Simulink" add-on.
      mask DialogControl exportToModel Prompt: Export
      mask DialogControl exportToModel Callback: exportConverterModelFromMask(gcb);
      mask Display:
      | llcModel = get_param(gcb, 'llcConverterModel');
      | rectOpt = get_param(gcb, 'rectifierOption');
      | if strcmp(llcModel, 'Detailed Full-Bridge')
      |     if strcmp(rectOpt, 'Full Bridge')
      |         image('FullBridgeLLCFullBridgeRectifier.svg', [0 0 1 1]);
      |     else
      |         image('FullBridgeLLCCentreTapRectifier.svg', [0 0 1 1]);
      |     end
      | else
      |     if strcmp(rectOpt, 'Full Bridge')
      |         image('HalfBridgeLLCFullBridgeRectifier.svg', [0 0 1 1]);
      |     else
      |         image('HalfBridgeLLCCentreTapRectifier.svg', [0 0 1 1]);
      |     end
      | end

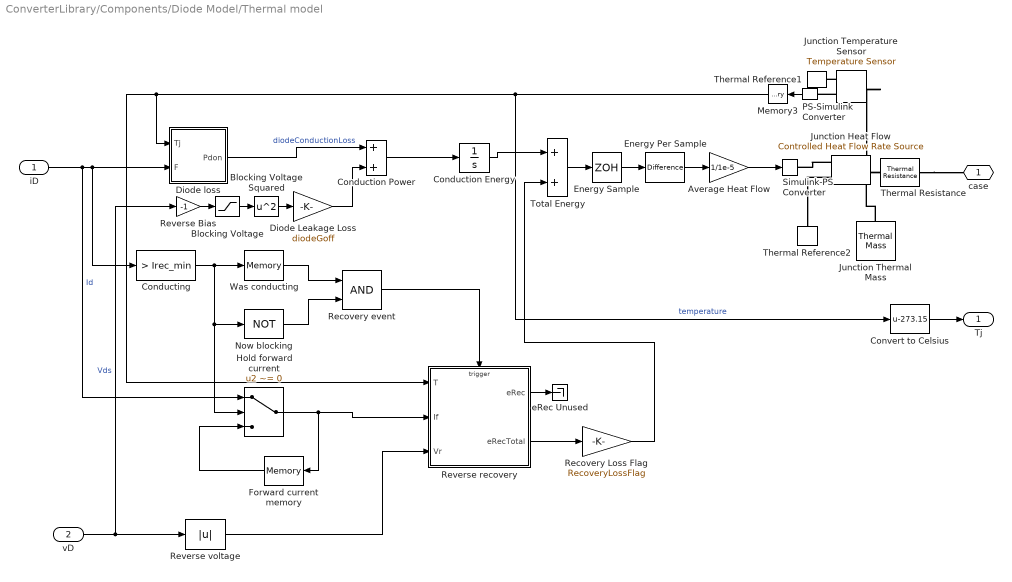
== system ConverterLibrary/Components/Diode Model/Thermal model ==
  iD : Inport
  vD : Inport  Port=2
  Average Heat Flow : Gain  Gain=1/1e-5
  Blocking Voltage : Saturate  UpperLimit=inf  LowerLimit=0
  Blocking Voltage Squared : Math  Operator=square
  Conducting : simulink/Logic and Bit Operations/Compare To Constant  relop=>  const=Irec_min  OutDataTypeStr=boolean
  Conduction Energy : Integrator
  Conduction Power : Sum
  Convert to Celsius : Bias  Bias=-273.15  SaturateOnIntegerOverflow=off
  Diode Leakage Loss : Gain  Gain=diodeGoff
  Diode loss : Subsystem
  Energy Per Sample : simulink/Discrete/Difference  ICPrevInput=0.0  OutMin=[]  OutMax=[]  OutDataType=fixdt(1, 16)  OutScaling=2^-10  DoSatur=off
  Energy Sample : ZeroOrderHold  SampleTime=1e-5
  Forward current memory : Memory
  Hold forward current : Switch  Criteria=u2 ~= 0  SaturateOnIntegerOverflow=off  InputSameDT=off
  Junction Heat Flow : fl_lib/Thermal/Thermal Sources/Controlled Heat Flow Rate Source
  Junction Temperature Sensor : fl_lib/Thermal/Thermal Sensors/Temperature Sensor  temperature_measure=foundation.enum.MeasurementReference.difference
  Junction Thermal Mass : fl_lib/Thermal/Thermal Elements/Thermal Mass  mass_type=foundation.enum.constant_variable.constant  mass=thermal_mass kg  sp_heat=1 J/(K*kg)  mass_min=1e-6 kg  num_ports=foundation.enum.numPorts2.one  m_specify=off  m_priority=High  m=1 kg  m_nominal_specify=off  m_nominal_value=1  m_nominal_unit=kg  T_specify=on  T_priority=High  T=Tj0 K  T_nominal_specify=off  T_nominal_value=1  T_nominal_unit=K  Q_specify=off  Q_priority=None  Q=0 W  Q_nominal_specify=off  Q_nominal_value=1  Q_nominal_unit=W
  Memory3 : Memory  InitialCondition=Tj0
  Now blocking : Logic  Operator=NOT  AllPortsSameDT=off  OutDataTypeStr=boolean
  PS-Simulink Converter : nesl_utility/PS-Simulink Converter  PhysicalDomain=network_engine_domain  SubClassName=ps_output  LeftPortType=input  RightPortType=output  PseudoPeriodic=off  Frequencies=[]  VectorFormat=inherit  Unit=K  AffineConversion=off
  Recovery Loss Flag : Gain  Gain=RecoveryLossFlag
  Recovery event : Logic  AllPortsSameDT=off  OutDataTypeStr=boolean
  Reverse Bias : Gain  Gain=-1
  Reverse recovery : Subsystem
  Reverse voltage : Abs  SaturateOnIntegerOverflow=off
  Simulink-PS Converter : nesl_utility/Simulink-PS Converter  PhysicalDomain=network_engine_domain  SubClassName=ps_input  LeftPortType=input  RightPortType=output  PseudoPeriodic=off  Frequencies=[]  NoiseDistribution=none  NoiseParameters=[]  Unit=W  AffineConversion=off  FilteringAndDerivatives=zero  SimscapeFilterOrder=1  InputFilterTimeConstant=0.001  UdotUserProvided=0
  Thermal Reference1 : fl_lib/Thermal/Thermal Elements/Thermal Reference
  Thermal Reference2 : fl_lib/Thermal/Thermal Elements/Thermal Reference
  Thermal Resistance : fl_lib/Thermal/Thermal Elements/Thermal Resistance  resistance=thermal_resistance K/W  T_specify=off  T_priority=None  T=0 K  T_nominal_specify=off  T_nominal_value=1  T_nominal_unit=K  Q_specify=off  Q_priority=None  Q=0 W  Q_nominal_specify=off  Q_nominal_value=1  Q_nominal_unit=W
  Total Energy : Sum
  Was conducting : Memory
  eRec Unused : Terminator
  case : PMIOPort  Side=Right
  Tj : Outport
  wires:
  Convert to Celsius/1 -> Tj/1
  Memory3/1 -> Reverse recovery/1(T), Diode loss/1(Tj), Convert to Celsius/1  "temperature"
  iD/1 -> Conducting/1, Diode loss/2(F), Hold forward current/1  "Id"
  Conducting/1 -> Now blocking/1, Hold forward current/2, Was conducting/1
  Was conducting/1 -> Recovery event/1
  Now blocking/1 -> Recovery event/2
  Hold forward current/1 -> Reverse recovery/2(If), Forward current memory/1
  Forward current memory/1 -> Hold forward current/3
  vD/1 -> Reverse voltage/1, Reverse Bias/1  "Vds"
  Reverse voltage/1 -> Reverse recovery/3(Vr)
  Recovery event/1 -> Reverse recovery/Trigger
  Reverse Bias/1 -> Blocking Voltage/1
  Blocking Voltage/1 -> Blocking Voltage Squared/1
  Blocking Voltage Squared/1 -> Diode Leakage Loss/1
  Diode loss/1(Pdon) -> Conduction Power/1  "diodeConductionLoss"
  Conduction Power/1 -> Conduction Energy/1
  Conduction Energy/1 -> Total Energy/1
  Reverse recovery/2(eRecTotal) -> Recovery Loss Flag/1
  Recovery Loss Flag/1 -> Total Energy/2
  Total Energy/1 -> Energy Sample/1
  Energy Sample/1 -> Energy Per Sample/1
  Energy Per Sample/1 -> Average Heat Flow/1
  Average Heat Flow/1 -> Simulink-PS Converter/1
  PS-Simulink Converter/1 -> Memory3/1
  Reverse recovery/1(eRec) -> eRec Unused/1
  Diode Leakage Loss/1 -> Conduction Power/2
  connections:
  Junction Heat Flow/LConn1 -- Thermal Resistance/RConn1 -- Junction Temperature Sensor/LConn1 -- Junction Thermal Mass/LConn1
  Junction Heat Flow/RConn1 -- Simulink-PS Converter/RConn1
  Junction Heat Flow/RConn2 -- Thermal Reference2/LConn1
  Junction Temperature Sensor/RConn1 -- Thermal Reference1/LConn1
  Junction Temperature Sensor/RConn2 -- PS-Simulink Converter/LConn1
  Thermal Resistance/LConn1 -- case/RConn1

== system ConverterLibrary/Components/IGBT Model/Antiparallel Diode ==
  ExternalDiode : Subsystem  VariantControl=ExternalDiode
  InbuiltDiode : Subsystem  VariantControl=InbuiltDiode
  P : PMIOPort  Side=Left
  N : PMIOPort  Port=2  Side=Left
  Id : Outport

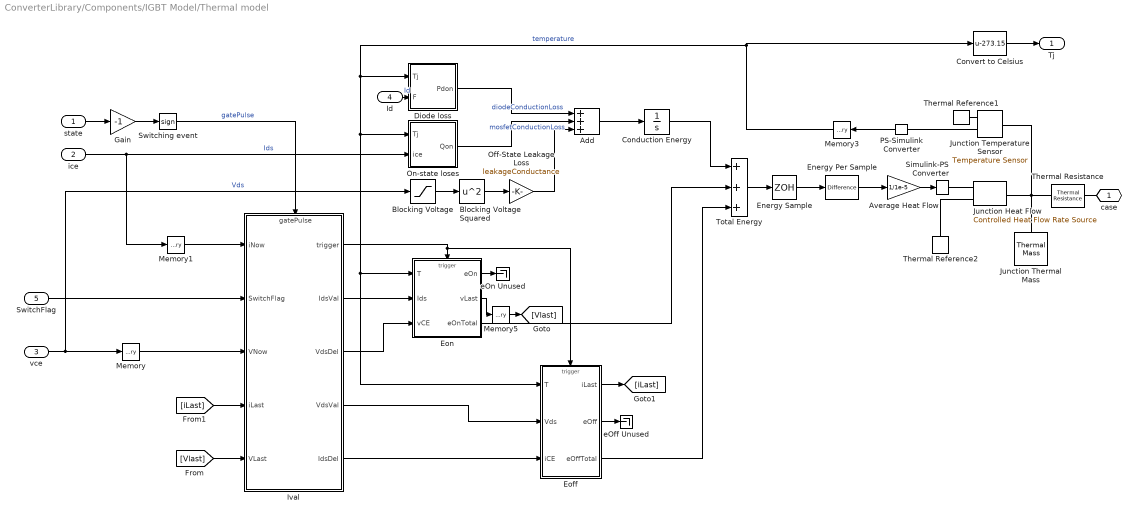
== system ConverterLibrary/Components/IGBT Model/Thermal model ==
  state : Inport
  ice : Inport  Port=2
  vce : Inport  Port=3
  Id : Inport  Port=4
  SwitchFlag : Inport  Port=5
  Add : Sum  Inputs=+++
  Average Heat Flow : Gain  Gain=1/1e-5
  Blocking Voltage : Saturate  UpperLimit=inf  LowerLimit=0
  Blocking Voltage Squared : Math  Operator=square
  Conduction Energy : Integrator
  Convert to Celsius : Bias  Bias=-273.15  SaturateOnIntegerOverflow=off
  Diode loss : Subsystem
  Energy Per Sample : simulink/Discrete/Difference  ICPrevInput=0.0  OutMin=[]  OutMax=[]  OutDataType=fixdt(1, 16)  OutScaling=2^-10  DoSatur=off
  Energy Sample : ZeroOrderHold  SampleTime=1e-5
  Eoff : Subsystem
  Eon : Subsystem
  Gain : Gain  Gain=-1
  Ival : Subsystem
      settings: PortSchema="{\"entries\":[{\"content\":{\"sides\":[{\"content\":{\"connectorIds\":[\"In1\",\"In2\",\"In3\",\"In4\",\"In5\"]},\"type\":\"ConnectorPlacement.EquallySpacedRectSide\",\"uuid\":\"a553ebc5-b0a0-4a8e-bff0-a68d2801e087\"},{\"content\":{\"connectorIds\":[\"Out1\",\"Out2\",\"Out3\",\"Out4\",\"Out5\"],\"side\":\"RIGHT\"},\"type\":\"ConnectorPlacement.EquallySpacedRectSide\",\"uuid\":\"ac80ac7d-324c-4908-a07c-53a421efec51\"},{\"content\":{\"connectorIds\":[\"In6\"],\"side\":\"TOP\"},\"type\":\"ConnectorPlacement.EquallySpacedRectSide\",\"uuid\":\"7840bf98-6f1a-4afc-8020-e550163e4138\"}]},\"type\":\"ConnectorPlacement.EquallySpacedConnector\",\"uuid\":\"bf4a6777-16de-4536-9449-5f030ac27c09\"}],\"packageUris\":[\"http://schema.mathworks.com/mf0/Connector/R2020b\"],\"version\":\"1.0\"}"
  Junction Heat Flow : fl_lib/Thermal/Thermal Sources/Controlled Heat Flow Rate Source
  Junction Temperature Sensor : fl_lib/Thermal/Thermal Sensors/Temperature Sensor  temperature_measure=foundation.enum.MeasurementReference.difference
  Junction Thermal Mass : fl_lib/Thermal/Thermal Elements/Thermal Mass  mass_type=foundation.enum.constant_variable.constant  mass=thermal_mass kg  sp_heat=1 J/(K*kg)  mass_min=1e-6 kg  num_ports=foundation.enum.numPorts2.one  m_specify=off  m_priority=High  m=1 kg  m_nominal_specify=off  m_nominal_value=1  m_nominal_unit=kg  T_specify=on  T_priority=High  T=Tj0 K  T_nominal_specify=off  T_nominal_value=1  T_nominal_unit=K  Q_specify=off  Q_priority=None  Q=0 W  Q_nominal_specify=off  Q_nominal_value=1  Q_nominal_unit=W
  Memory : Memory  InitialCondition=Voff
  Memory1 : Memory
  Memory3 : Memory  InitialCondition=Tj0
  Memory5 : Memory
  Off-State Leakage Loss : Gain  Gain=leakageConductance
  On-state loses : Subsystem
  PS-Simulink Converter : nesl_utility/PS-Simulink Converter  PhysicalDomain=network_engine_domain  SubClassName=ps_output  LeftPortType=input  RightPortType=output  PseudoPeriodic=off  Frequencies=[]  VectorFormat=inherit  Unit=K  AffineConversion=off
  Simulink-PS Converter : nesl_utility/Simulink-PS Converter  PhysicalDomain=network_engine_domain  SubClassName=ps_input  LeftPortType=input  RightPortType=output  PseudoPeriodic=off  Frequencies=[]  NoiseDistribution=none  NoiseParameters=[]  Unit=W  AffineConversion=off  FilteringAndDerivatives=zero  SimscapeFilterOrder=1  InputFilterTimeConstant=0.001  UdotUserProvided=0
  Switching event : Signum
  Thermal Reference1 : fl_lib/Thermal/Thermal Elements/Thermal Reference
  Thermal Reference2 : fl_lib/Thermal/Thermal Elements/Thermal Reference
  Thermal Resistance : fl_lib/Thermal/Thermal Elements/Thermal Resistance  resistance=thermal_resistance K/W  T_specify=off  T_priority=None  T=0 K  T_nominal_specify=off  T_nominal_value=1  T_nominal_unit=K  Q_specify=off  Q_priority=None  Q=0 W  Q_nominal_specify=off  Q_nominal_value=1  Q_nominal_unit=W
  Total Energy : Sum  Inputs=+++
  eOff Unused : Terminator
  eOn Unused : Terminator
  case : PMIOPort  Side=Right
  Tj : Outport
  wires:
  ice/1 -> On-state loses/2(ice), Memory1/1  "Ids"
  Switching event/1 -> Ival/6(gatePulse)  "gatePulse"
  Memory1/1 -> Ival/1(iNow)
  Eon/2(vLast) -> Memory5/1
  Convert to Celsius/1 -> Tj/1
  state/1 -> Gain/1
  vce/1 -> Memory/1, Blocking Voltage/1  "Vds"
  Id/1 -> Diode loss/2(F)  "Id"
  SwitchFlag/1 -> Ival/2(SwitchFlag)
  Memory5/1 -> [Vlast]
  Eoff/1(iLast) -> [iLast]
  Gain/1 -> Switching event/1
  [iLast] -> Ival/4(iLast)
  Ival/4(VdsVal) -> Eoff/2(Vds)
  Ival/1(trigger) -> Eoff/Trigger, Eon/Trigger
  [Vlast] -> Ival/5(VLast)
  Memory/1 -> Ival/3(VNow)
  Ival/2(IdsVal) -> Eon/2(Ids)
  Ival/3(VdsDel) -> Eon/3(vCE)
  Ival/5(IdsDel) -> Eoff/3(iCE)
  On-state loses/1(Qon) -> Add/2  "mosfetConductionLoss"
  Add/1 -> Conduction Energy/1
  Total Energy/1 -> Energy Sample/1
  Energy Sample/1 -> Energy Per Sample/1
  Energy Per Sample/1 -> Average Heat Flow/1
  Average Heat Flow/1 -> Simulink-PS Converter/1
  PS-Simulink Converter/1 -> Memory3/1
  Eon/1(eOn) -> eOn Unused/1
  Eoff/2(eOff) -> eOff Unused/1
  Memory3/1 -> Convert to Celsius/1, Diode loss/1(Tj), On-state loses/1(Tj), Eon/1(T), Eoff/1(T)  "temperature"
  Conduction Energy/1 -> Total Energy/1
  Eon/3(eOnTotal) -> Total Energy/2
  Eoff/3(eOffTotal) -> Total Energy/3
  Diode loss/1(Pdon) -> Add/1  "diodeConductionLoss"
  Blocking Voltage/1 -> Blocking Voltage Squared/1
  Blocking Voltage Squared/1 -> Off-State Leakage Loss/1
  Off-State Leakage Loss/1 -> Add/3
  connections:
  case/RConn1 -- Thermal Resistance/LConn1
  Junction Heat Flow/LConn1 -- Junction Thermal Mass/LConn1 -- Thermal Resistance/RConn1 -- Junction Temperature Sensor/LConn1
  Junction Heat Flow/RConn1 -- Simulink-PS Converter/RConn1
  Junction Heat Flow/RConn2 -- Thermal Reference2/LConn1
  Junction Temperature Sensor/RConn1 -- Thermal Reference1/LConn1
  Junction Temperature Sensor/RConn2 -- PS-Simulink Converter/LConn1
